simulink model "ContModelHIL"  (R2026a)
settings: Solver=ode4  StopTime=inf  FixedStep=0.01  EnableMultiTasking=on
PreLoadFcn:
  | init_var;
values from neighbouring files (symbols this model uses):
  Observer = struct('E1', E1 ,     'E2', E2 ,     'E3', E3 ,     'E4', E4 ,     'MU1', MU1 ,     'MU2', MU2 ,     'MU3', MU3 ,     'alpha', alpha ,     'beta', beta)    [init_model.m]    (also in init_var.m)
  PID = InitController()    [init_model.m]    (also in init_var.m)
  st = 0.01    [init_model.m]    (also in init_var.m; px4HostTarget_TCPIP_Read.m = matlab.system.SampleTimeSpecification('Type', 'Discrete',   )
undefined symbols (not defined in the file or in its folder): DiscIntNeverNeededParam
libraries: px4Peripheralslib x1, px4uORBlib x1
settings Model: ExtModeTrigDuration=10  Creator=Carlos Fabian  LastModifiedBy=Carlos Fabian
settings SolverCC: PositivePriorityOrder=on
settings HardwareCC: ProdLargestAtomicInteger=Long  ProdLargestAtomicFloat=Double  ProdHWDeviceType=ARM Compatible->ARM Cortex
settings SFSimCC: SimTargetLang=C++
settings RTWCC: SystemTargetFile=ert.tlc  HardwareBoard=PX4 Pixhawk 6c  TLCOptions="-aInlineSetEventsForThisBaseRateFcn=TLC_FALSE -aSuppressMultiTaskScheduler=TLC_FALSE  -aRateBasedStepFcn=0"  Toolchain=GNU Tools for PX4 Autopilots  TargetLang=C++  Description=Embedded Coder
settings ERTTargetCC: ExtModeTransport=3.0  ExtModeStaticAllocSize=1024.0
settings ExplorerConfigSet: InternalSimMechanicsExplorerSettings=|
  | <ExplorerConfiguration>
  | 
  |   <canonicalview>default</canonicalview>
  | 
  |   <TilePanel>
  |     <TileInfo>
  |       <Tiles Columns="1" Count="1" Height="513" Rows="1" Width="774">
  |         <Row Weight="1"/>
  |         <Column Weight="1"/>
  |         <Tile Height="1" Width="1" X="0" Y="0"/>
  |       </Tiles>
  |     </TileInfo>
  |     <SceneInfo>
  |       <SceneViewer>
  |         <IsThisViewStd>
  |           <IsStandardView>off</IsStandardView>
  |           <StandardViewName>Front</StandardViewName>
  |         </IsThisViewStd>
  |         <BGColor>
  |           <R>1</R>
  |           <G>1</G>
  |           <B>1</B>
  |           <A>1</A>
  |         </BGColor>
  |         <Camera>
  |           <DoPerspective>off</DoPerspective>
  |           <Position>
  |             <X>16.201091586104312</X>
  |             <Y>-16.65504514146788</Y>
  |             <Z>17.087073385082522</Z>
  |           </Position>
  |           <Center>
  |             <X>-0.25720946651222221</X>
  |             <Y>-0.19674408885134653</Y>
  |             <Z>0.62877233246599318</Z>
  |           </Center>
  |           <Up>
  |             <X>-0.40824829046386302</X>
  |             <Y>0.40824829046386302</Y>
  |             <Z>0.81649658092772615</Z>
  |           </Up>
  |           <XLim>2.5491252053936631</XLim>
  |           <YLim>2.5491252053936631</YLim>
  |           <ViewLimDist>0.01</ViewLimDist>
  |         </Camera>
  |       </SceneViewer>
  |     </SceneInfo>
  |   </TilePanel>
  | 
  |   <MechEditorPanel>
  |     <GfxPanelCameraMap/>
  |     <Cameras/>
  |     <VideoCreator>
  |       <IncludeTiles>All</IncludeTiles>
  |       <IncludeTime>on</IncludeTime>
  |       <IncludeWorldFrame>off</IncludeWorldFrame>
  |       <PlaybackSpeedRatio>8</PlaybackSpeedRatio>
  |       <FrameRate>24</FrameRate>
  |       <FrameSize>auto</FrameSize>
  |       <VideoFormat>MotionJPEGAVI</VideoFormat>
  |     </VideoCreator>
  |   </MechEditorPanel>
  | 
  |   <PlaybackSettings>
  |     <PlaybackSpeedFactor>16</PlaybackSpeedFactor>
  |   </PlaybackSettings>
  | 
  | </ExplorerConfiguration>

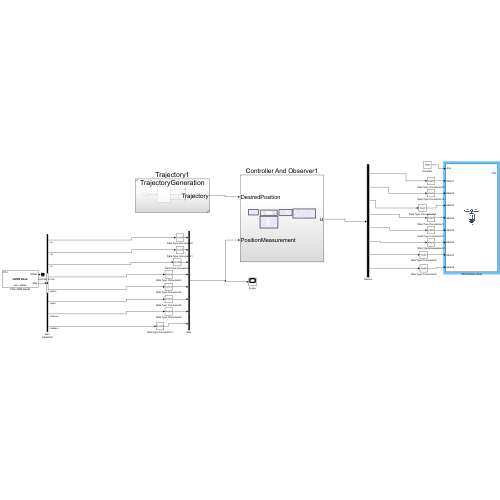
[thumbnail: Simulink's stored preview of the top-level diagram]
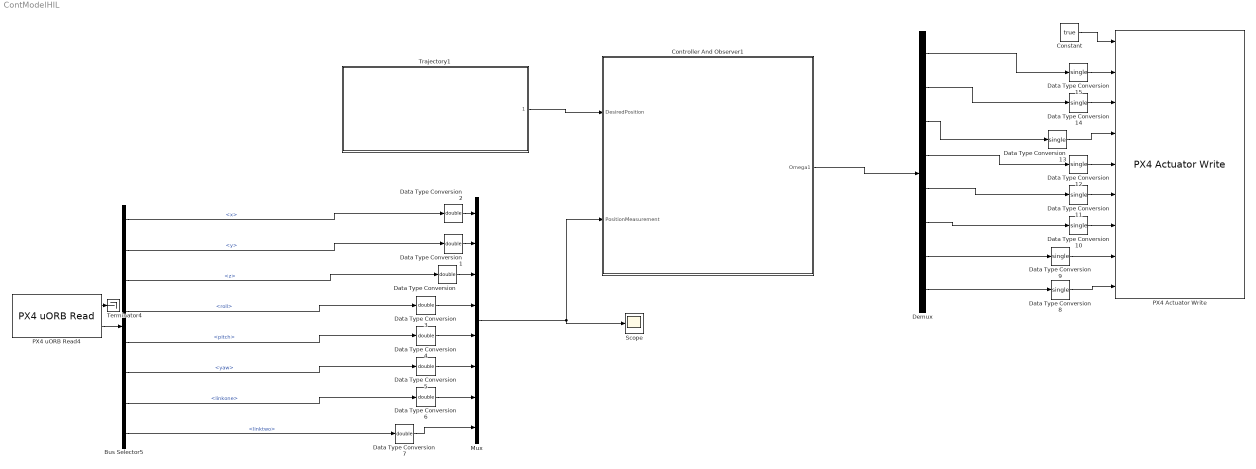
== system ContModelHIL ==
  Bus Selector5 : BusSelector  OutputSignals=x,y,z,roll,pitch,yaw,linkone,linktwo
  Constant : Constant  Value=true
  Controller And Observer1 : Subsystem
  Data Type Conversion{,1..7} (8 alike) : DataTypeConversion  OutDataTypeStr=double  SaturateOnIntegerOverflow=off  RndMeth=Floor
  Data Type Conversion{8..15} (8 alike) : DataTypeConversion  OutDataTypeStr=single  SaturateOnIntegerOverflow=off  RndMeth=Floor
  Demux : Demux  Outputs=8
  Mux : Mux  Inputs=8
  PX4 Actuator Write : px4Peripheralslib/PX4 Actuator Write  Motor1Enable=on  Motor2Enable=on  Motor3Enable=on  Motor4Enable=on  Motor5Enable=on  Motor6Enable=on  Motor7Enable=on  Motor8Enable=on  Motor9Enable=off  Motor10Enable=off  Motor11Enable=off  Motor12Enable=off  IsMotorArray=off  Servo1Enable=off  Servo2Enable=off  Servo3Enable=off  Servo4Enable=off  Servo5Enable=off  Servo6Enable=off  Servo7Enable=off  Servo8Enable=off  IsServoArray=off
  PX4 uORB Read4 : px4uORBlib/PX4 uORB Read  uORBMsg=UamStates  uORBTopicName=uam_states  SubscribeNonZeroInstance=off  selectInstanceNum=1  SampleTime=0.01  isSingleTopicMsg=on  BlockingMode=off  BlockTimeout=1e-3
  Scope : Scope
      settings: ActiveDisplayYMinimum=-24.375562229014246  ActiveDisplayYMaximum=17.203001359213125
  Terminator4 : Terminator
  Trajectory1 : Subsystem  ReferencedSubsystem=TrajectoryGeneration
  wires:
  Trajectory1/1 -> Controller And Observer1/1(DesiredPosition)
  Bus Selector5/7 -> Data Type Conversion6/1  "<linkone>"
  Bus Selector5/8 -> Data Type Conversion7/1  "<linktwo>"
  Mux/1 -> Scope/1, Controller And Observer1/2(PositionMeasurement)
  Data Type Conversion/1 -> Mux/3
  Data Type Conversion1/1 -> Mux/2
  Data Type Conversion2/1 -> Mux/1
  Data Type Conversion3/1 -> Mux/4
  Data Type Conversion4/1 -> Mux/5
  Data Type Conversion5/1 -> Mux/6
  Data Type Conversion6/1 -> Mux/7
  Data Type Conversion7/1 -> Mux/8
  Data Type Conversion8/1 -> PX4 Actuator Write/9
  Data Type Conversion9/1 -> PX4 Actuator Write/8
  Data Type Conversion10/1 -> PX4 Actuator Write/7
  ? -> ?
  Data Type Conversion11/1 -> PX4 Actuator Write/6
  Data Type Conversion12/1 -> PX4 Actuator Write/5
  Data Type Conversion13/1 -> PX4 Actuator Write/4
  Data Type Conversion14/1 -> PX4 Actuator Write/3
  Data Type Conversion15/1 -> PX4 Actuator Write/2
  PX4 uORB Read4/2 -> Bus Selector5/1
  PX4 uORB Read4/1 -> Terminator4/1
  Bus Selector5/1 -> Data Type Conversion2/1  "<x>"
  Bus Selector5/2 -> Data Type Conversion1/1  "<y>"
  Bus Selector5/3 -> Data Type Conversion/1  "<z>"
  Bus Selector5/4 -> Data Type Conversion3/1  "<roll>"
  Bus Selector5/5 -> Data Type Conversion4/1  "<pitch>"
  Bus Selector5/6 -> Data Type Conversion5/1  "<yaw>"
  Controller And Observer1/1(Omega1) -> Demux/1
  Demux/1 -> Data Type Conversion15/1
  Demux/2 -> Data Type Conversion14/1
  Demux/3 -> Data Type Conversion13/1
  Demux/4 -> Data Type Conversion12/1
  Demux/5 -> Data Type Conversion11/1
  Demux/6 -> Data Type Conversion10/1
  Demux/7 -> Data Type Conversion9/1
  Demux/8 -> Data Type Conversion8/1
  Constant/1 -> PX4 Actuator Write/1

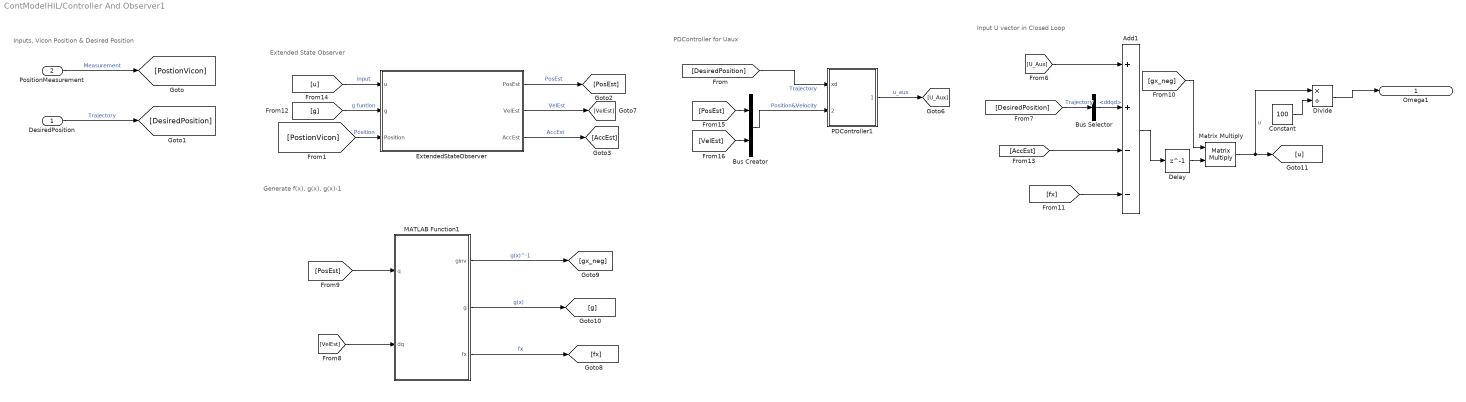
== system ContModelHIL/Controller And Observer1 ==
  note: Extended State Observer
  note: Input U vector in Closed Loop
  note: Generate f(x), g(x), g(x)-1
  note: PDController for Uaux
  note: Inputs, Vicon Position & Desired Position
  DesiredPosition : Inport
  PositionMeasurement : Inport  Port=2
  Add1 : Sum  Inputs=++--
  Bus Creator : BusCreator  Inputs=2
  Bus Selector : BusSelector  OutputSignals=ddqd
  Constant : Constant  Value=100
  Delay : Delay  DelayLength=1  InitialCondition=0
  Divide : Product  Inputs=*/
  ExtendedStateObserver : Subsystem
  MATLAB Function1 : MATLAB Function  TreatAsAtomicUnit=on
  Matrix Multiply : Product  Multiplication=Matrix(*)
  PDController1 : Subsystem
  Omega1 : Outport
  wires:
  [PostionVicon] -> ExtendedStateObserver/3(Position)  "Position"
  [DesiredPosition] -> PDController1/1(xd)  "Trajectory"
  ExtendedStateObserver/1(PosEst) -> [PosEst]  "PosEst"
  PositionMeasurement/1 -> [PostionVicon]  "Measurement"
  DesiredPosition/1 -> [DesiredPosition]  "Trajectory"
  Bus Creator/1 -> PDController1/2(q_hat1)  "Position&Velocity"
  ExtendedStateObserver/3(AccEst) -> [AccEst]  "AccEst"
  ExtendedStateObserver/2(VelEst) -> [VelEst]  "VelEst"
  PDController1/1(Output) -> [U_Aux]  "u_aux"
  MATLAB Function1/1(ginv) -> [gx_neg]  "g(x)^-1"
  MATLAB Function1/3(fx) -> [fx]  "fx"
  Add1/1 -> Delay/1
  Matrix Multiply/1 -> Divide/1, [u]  "u"
  [DesiredPosition] -> Bus Selector/1  "Trajectory"
  Bus Selector/1 -> Add1/2  "<ddqd>"
  MATLAB Function1/2(g) -> [g]  "g(x)"
  [PosEst] -> Bus Creator/1
  [VelEst] -> Bus Creator/2
  [u] -> ExtendedStateObserver/1(u)  "input"
  [g] -> ExtendedStateObserver/2(g)  "g funtion"
  [PosEst] -> MATLAB Function1/1(q)
  [VelEst] -> MATLAB Function1/2(dq)
  [fx] -> Add1/4
  [gx_neg] -> Matrix Multiply/1
  [U_Aux] -> Add1/1
  [AccEst] -> Add1/3
  Delay/1 -> Matrix Multiply/2
  Divide/1 -> Omega1/1
  Constant/1 -> Divide/2

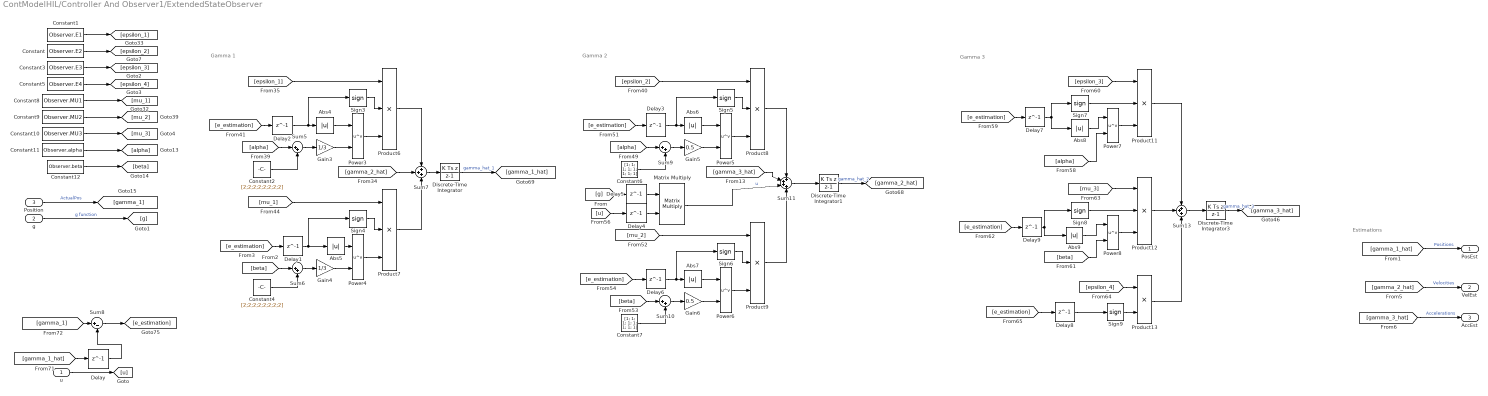
== system ContModelHIL/Controller And Observer1/ExtendedStateObserver ==
  note: Estimations
  note: Gamma 3
  note: Gamma 2
  note: Gamma 1
  u : Inport
  g : Inport  Port=2
  Position : Inport  Port=3
  Abs{4..9} (6 alike) : Abs  SaturateOnIntegerOverflow=off
  Constant : Constant  Value=Observer.E2
  Constant1 : Constant  Value=Observer.E1
  Constant10 : Constant  Value=Observer.MU3
  Constant11 : Constant  Value=Observer.alpha
  Constant12 : Constant  Value=Observer.beta
  Constant2 : Constant  Value=[2;2;2;2;2;2;2;2]
  Constant3 : Constant  Value=Observer.E3
  Constant4 : Constant  Value=[2;2;2;2;2;2;2;2]
  Constant5 : Constant  Value=Observer.E4
  Constant6 : Constant  Value=[1; 1; 1; 1; 1; 1; 1; 1]
  Constant7 : Constant  Value=[1; 1; 1; 1; 1; 1; 1; 1]
  Constant8 : Constant  Value=Observer.MU1
  Constant9 : Constant  Value=Observer.MU2
  Delay{,1..9} (10 alike) : Delay  DelayLength=1  InitialCondition=0  SampleTime=0.01
  Discrete-Time Integrator : DiscreteIntegrator  IntegratorMethod=Integration: Backward Euler  InitialCondition=[0; 0; 0.24; 0; 0; 0; 0; 0]  SampleTime=st  ICPrevOutput=DiscIntNeverNeededParam  ICPrevScaledInput=DiscIntNeverNeededParam
  Discrete-Time Integrator1 : DiscreteIntegrator  IntegratorMethod=Integration: Backward Euler  InitialCondition=zeros(8,1)  SampleTime=st  ICPrevOutput=DiscIntNeverNeededParam  ICPrevScaledInput=DiscIntNeverNeededParam
  Discrete-Time Integrator3 : DiscreteIntegrator  IntegratorMethod=Integration: Backward Euler  InitialCondition=[0; 0; -9.81; 0; 0; 0; 0; 0]  SampleTime=st  ICPrevOutput=DiscIntNeverNeededParam  ICPrevScaledInput=DiscIntNeverNeededParam
  Gain3 : Gain  Gain=1/3
  Gain4 : Gain  Gain=1/3
  Gain5 : Gain  Gain=0.5
  Gain6 : Gain  Gain=0.5
  Matrix Multiply : Product  Multiplication=Matrix(*)
  Power{3..8} (6 alike) : Math  Operator=pow
  Product{6..9,11..12} (6 alike) : Product  Inputs=3
  Product13 : Product
  Sign{3..9} (7 alike) : Signum
  Sum{5..6,9..10} (4 alike) : Sum  Inputs=|++
  Sum11 : Sum  Inputs=++++
  Sum13 : Sum  Inputs=+++
  Sum7 : Sum  Inputs=+++
  Sum8 : Sum  Inputs=|+-
  PosEst : Outport
  VelEst : Outport  Port=2
  AccEst : Outport  Port=3
  wires:
  Constant11/1 -> [alpha]
  [beta] -> Sum10/1
  [e_estimation] -> Delay9/1
  Power7/1 -> Product11/3
  Matrix Multiply/1 -> Sum11/3  "u"
  Constant12/1 -> [beta]
  [e_estimation] -> Delay7/1
  [gamma_1_hat] -> PosEst/1  "Positions"
  Power8/1 -> Product12/3
  Constant4/1 -> Sum6/2
  [alpha] -> Sum5/1
  Product6/1 -> Sum7/1
  Abs8/1 -> Power7/1
  Power5/1 -> Product8/3
  [gamma_1] -> Sum8/1
  [e_estimation] -> Delay6/1
  [epsilon_2] -> Product8/1
  Sum11/1 -> Discrete-Time Integrator1/1
  Constant10/1 -> [mu_3]
  Gain5/1 -> Power5/2
  [e_estimation] -> Delay2/1
  Abs5/1 -> Power4/1
  Sum13/1 -> Discrete-Time Integrator3/1
  Abs7/1 -> Power6/1
  Product9/1 -> Sum11/4
  [epsilon_1] -> Product6/1
  Constant7/1 -> Sum10/2
  [epsilon_3] -> Product11/1
  Sum9/1 -> Gain5/1
  Sum6/1 -> Gain4/1
  [e_estimation] -> Delay3/1
  u/1 -> [u]
  [mu_3] -> Product12/1
  Sign6/1 -> Product9/2
  Sum7/1 -> Discrete-Time Integrator/1
  Sign8/1 -> Product12/2
  [alpha] -> Power7/2
  [epsilon_4] -> Product13/1
  [gamma_3_hat] -> Sum11/2
  [mu_1] -> Product7/1
  Sign3/1 -> Product6/2
  Discrete-Time Integrator1/1 -> [gamma_2_hat]  "gamma_hat_2"
  Constant/1 -> [epsilon_2]
  [mu_2] -> Product9/1
  Product11/1 -> Sum13/1
  Sign4/1 -> Product7/2
  Product7/1 -> Sum7/3
  Constant9/1 -> [mu_2]
  Constant1/1 -> [epsilon_1]
  Constant6/1 -> Sum9/2
  Sign5/1 -> Product8/2
  [beta] -> Power8/2
  Constant2/1 -> Sum5/2
  Gain6/1 -> Power6/2
  Gain3/1 -> Power3/2
  Power6/1 -> Product9/3
  Position/1 -> [gamma_1]  "ActualPos"
  Constant5/1 -> [epsilon_4]
  Constant3/1 -> [epsilon_3]
  Product13/1 -> Sum13/3
  Discrete-Time Integrator/1 -> [gamma_1_hat]  "gamma_hat_1"
  Sum5/1 -> Gain3/1
  Power3/1 -> Product6/3
  Power4/1 -> Product7/3
  Sum10/1 -> Gain6/1
  [gamma_2_hat] -> Sum7/2
  Sign7/1 -> Product11/2
  [beta] -> Sum6/1
  [e_estimation] -> Delay1/1
  [e_estimation] -> Delay8/1
  Product8/1 -> Sum11/1
  Sign9/1 -> Product13/2
  Abs9/1 -> Power8/1
  [alpha] -> Sum9/1
  Discrete-Time Integrator3/1 -> [gamma_3_hat]  "gamma_hat_3"
  Sum8/1 -> [e_estimation]
  Gain4/1 -> Power4/2
  Constant8/1 -> [mu_1]
  Product12/1 -> Sum13/2
  g/1 -> [g]  "g function"
  Abs6/1 -> Power5/1
  Abs4/1 -> Power3/1
  [gamma_3_hat] -> AccEst/1  "Accelerations"
  [gamma_2_hat] -> VelEst/1  "Velocities"
  [g] -> Delay5/1
  [u] -> Delay4/1
  [gamma_1_hat] -> Delay/1
  Delay/1 -> Sum8/2
  Delay1/1 -> Sign4/1, Abs5/1
  Delay2/1 -> Sign3/1, Abs4/1
  Delay3/1 -> Sign5/1, Abs6/1
  Delay4/1 -> Matrix Multiply/2
  Delay5/1 -> Matrix Multiply/1
  Delay6/1 -> Sign6/1, Abs7/1
  Delay7/1 -> Abs8/1, Sign7/1
  Delay8/1 -> Sign9/1
  Delay9/1 -> Sign8/1, Abs9/1

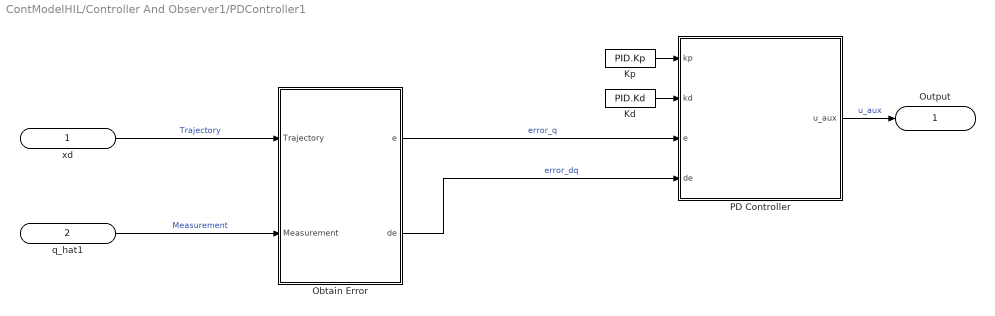
== system ContModelHIL/Controller And Observer1/PDController1 ==
  xd : Inport
  q_hat1 : Inport  Port=2
  Kd : Constant  Value=PID.Kd
  Kp : Constant  Value=PID.Kp
  Obtain Error : Subsystem
  PD Controller : MATLAB Function  TreatAsAtomicUnit=on
  Output : Outport
  wires:
  xd/1 -> Obtain Error/1(Trajectory)  "Trajectory"
  q_hat1/1 -> Obtain Error/2(Measurement)  "Measurement"
  Obtain Error/1(e) -> PD Controller/3(e)  "error_q"
  Obtain Error/2(de) -> PD Controller/4(de)  "error_dq"
  Kp/1 -> PD Controller/1(kp)
  Kd/1 -> PD Controller/2(kd)
  PD Controller/1(u_aux) -> Output/1  "u_aux"

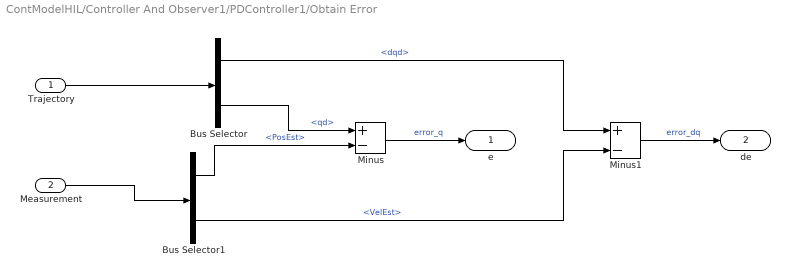
== system ContModelHIL/Controller And Observer1/PDController1/Obtain Error ==
  Trajectory : Inport
  Measurement : Inport  Port=2
  Bus Selector : BusSelector  OutputSignals=dqd,qd
  Bus Selector1 : BusSelector  OutputSignals=PosEst,VelEst
  Minus : Sum  Inputs=+-
  Minus1 : Sum  Inputs=+-
  e : Outport
  de : Outport  Port=2
  wires:
  Bus Selector1/1 -> Minus/2  "<PosEst>"
  Bus Selector1/2 -> Minus1/2  "<VelEst>"
  Measurement/1 -> Bus Selector1/1
  Trajectory/1 -> Bus Selector/1
  Bus Selector/1 -> Minus1/1  "<dqd>"
  Bus Selector/2 -> Minus/1  "<qd>"
  Minus/1 -> e/1  "error_q"
  Minus1/1 -> de/1  "error_dq"

== matlab function ContModelHIL/Controller And Observer1/MATLAB Function1 ==
  data: q input; dq input; ginv output; g output; fx output
function [ginv, g, fx] = Get_DCG_Hexa(q, dq)

DM = DFunMatrix(q);
CM = CFunMatrix(q, dq);
Gv = GFunVector(q);

g = inv(DM);
ginv = DM;

fx = DM\( -CM*dq - Gv );

end

== matlab function ContModelHIL/Controller And Observer1/PDController1/PD Controller ==
  data: kp input; kd input; u_aux output; e input; de input
function u_aux = pd_cont(kp, kd, e, de)


kp_m = [kp(1) 0       0     0     0       0     0     0;
        0     kp(2)   0     0     0       0     0     0;
        0     0       kp(3) 0     0       0     0     0;
        0     0       0     kp(4) 0       0     0     0;
        0     0       0     0     kp(5)   0     0     0;
        0     0       0     0     0       kp(6) 0     0;
        0     0       0     0     0       0     kp(7) 0;
        0     0       0     0     0       0     0     kp(8)];

kd_m = [kd(1) 0       0     0     0       0     0     0;
        0     kd(2)   0     0     0       0     0     0;
        0     0       kd(3) 0     0       0     0     0;
        0     0       0     kd(4) 0       0     0     0;
        0     0       0     0     kd(5)   0     0     0;
        0     0       0     0     0       kd(6) 0     0;
        0     0       0     0     0       0     kd(7) 0;
        0     0       0     0     0       0     0     kd(8)];


%v = ddP + kp_m * e + kd_m * de;
u_aux = kp_m * e + kd_m * de;
%v = ddP;

end
